simulink model "MPPT_PO1"  (R2024b)
settings: Solver=ode45  StartTime=0.0  StopTime=10.0  MaxStep=1e-4  RelTol=1e-3
libraries: powerlib_extras x2, simulink x1, spspowerguiLib x1
settings Model: Creator=Abdo  LastModifiedBy=Eng.Abd-Elrhman Saad
settings SolverCC: ZeroCrossAlgorithm=Adaptive  AlgebraicLoopSolver=TrustRegion
settings DataIOCC: SaveFormat=StructureWithTime  ReturnWorkspaceOutputs=off
settings OptimizationCC: LifeSpan=inf
settings DebuggingCC: MaxConsecutiveZCsMsg=none  UnconnectedInputMsg=warning  UnconnectedOutputMsg=warning  UnconnectedLineMsg=warning  SFExecutionAtInitializationDiag=none  ArithmeticOperatorsInVariantConditions=warning
settings HardwareCC: ProdBitPerSizeT=32  ProdBitPerPtrDiffT=32  ProdWordSize=32  ProdHWDeviceType=Specified
settings SFSimCC: SimUseLocalCustomCode=off  CustomCodeUndefinedFunction=UseInterfaceOnly
settings RTWCC: RTWUseLocalCustomCode=off  GPUComputeCapability=3.5
settings CodeAppCC: StateflowObjectComments=on

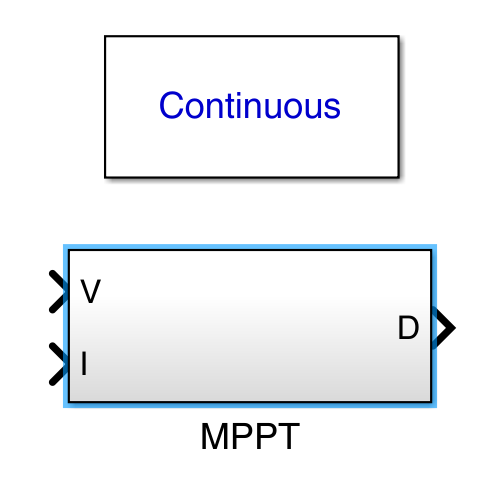
[thumbnail: Simulink's stored preview of the top-level diagram]
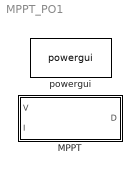
== system MPPT_PO1 ==
  MPPT : Subsystem
  powergui : spspowerguiLib/powergui  Priority=1  SimulationMode=Continuous  SampleTime=50e-6  frequency=60  Iterations=50  frequencyindice=0  Pbase=100e6  ErrMax=1e-4  UnitsV=kV  UnitsW=MW  buscounter=0  FunctionMessages=off  echomessages=off  EnableUseOfTLC=off  CurrentSourceSwitches=off  DisableSnubberDevices=off  DisableRonSwitches=off  DisableVfSwitches=off  DisplayEquations=off  AutomaticDiscreteSolvers=off  SolverType=Tustin/Backward Euler (TBE)  Interpol=off  ExternalGateDelay=off  methode=off  Ts=100  x0status=blocks  SPID=on  SwTol=0  HookPort=off  NonlinearTolerance=1e-4  nMaxIteration=100  ContinueOnMaxIteration=off  RestoreLinks=warning  ResistiveCurrentMeasurement=off  Frange=[0:2:500]  Ylog=off  Xlog=on  ShowGrid=off  save=off  variable=ZData  structure=0  ZoomFFT=off  StartTime=0.0  cycles=1  DisplayStyle=1  fundamental=60  FreqAxis=off  MaxFrequency=1000  frequencyindicesteady=1  RmsSteady=1  display=off

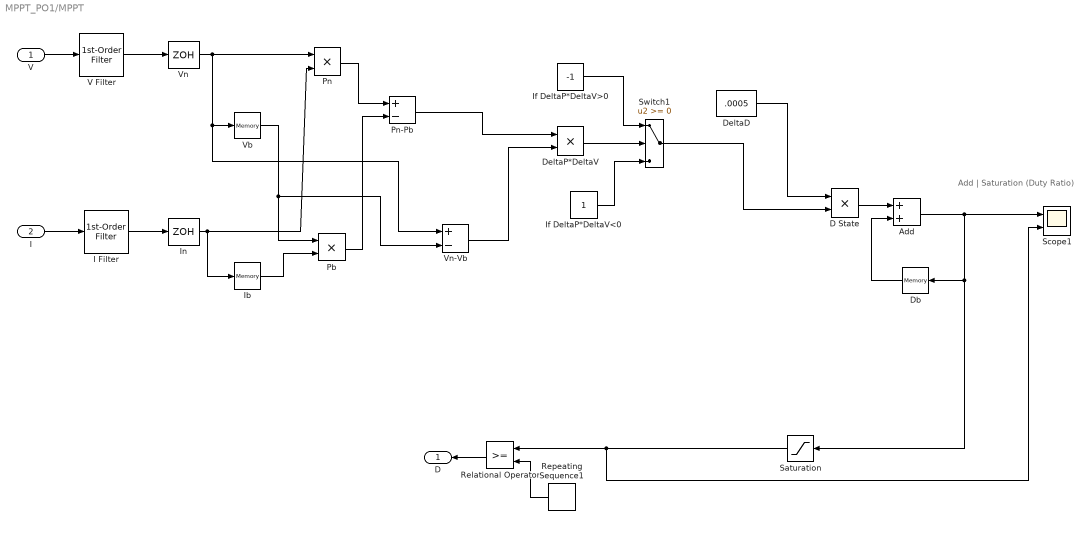
== system MPPT_PO1/MPPT ==
  note: Add | Saturation (Duty Ratio)
  V : Inport
  I : Inport  Port=2
  Add : Sum
  D State : Product  RndMeth=Zero
  Db : Memory  InheritSampleTime=on  LinearizeAsDelay=on
  DeltaD : Constant  Value=.0005
  DeltaP*DeltaV : Product  RndMeth=Zero
  I Filter : powerlib_extras/Control  Blocks/1st-Order  Filter  FilterType=Lowpass  Tc=1e-3  Initialize=off  Vac_Init=[0.8 -25 60]  Vdc_Init=-0.4  PlotResponse=off  param1=[1 500 1]
  Ib : Memory  InheritSampleTime=on  LinearizeAsDelay=on
  If DeltaP*DeltaV<0 : Constant
  If DeltaP*DeltaV>0 : Constant  Value=-1
  In : ZeroOrderHold  SampleTime=1e-4
  Pb : Product  RndMeth=Zero
  Pn : Product  RndMeth=Zero
  Pn-Pb : Sum  Inputs=+-
  Relational Operator : RelationalOperator  OutDataTypeStr=boolean  InputSameDT=off
  Repeating Sequence1 : simulink/Sources/Repeating Sequence  rep_seq_t=[0 1e-3]  rep_seq_y=[0 1]
  Saturation : Saturate  UpperLimit=0.9  LowerLimit=0
  Scope1 : Scope  NumInputPorts=2
  Switch1 : Switch  SaturateOnIntegerOverflow=off  InputSameDT=off
  V Filter : powerlib_extras/Control  Blocks/1st-Order  Filter  FilterType=Lowpass  Tc=1e-3  Initialize=off  Vac_Init=[0.8 -25 60]  Vdc_Init=-0.4  PlotResponse=off  param1=[1 500 1]
  Vb : Memory  InheritSampleTime=on  LinearizeAsDelay=on
  Vn : ZeroOrderHold  SampleTime=1e-4
  Vn-Vb : Sum  Inputs=+-
  D : Outport
  wires:
  V/1 -> V Filter/1
  I/1 -> I Filter/1
  V Filter/1 -> Vn/1
  I Filter/1 -> In/1
  In/1 -> Ib/1, Pn/2
  Vn/1 -> Pn/1, Vb/1, Vn-Vb/1
  Ib/1 -> Pb/2
  Vb/1 -> Pb/1, Vn-Vb/2
  Pn/1 -> Pn-Pb/1
  Pb/1 -> Pn-Pb/2
  D State/1 -> Add/1
  Repeating Sequence1/1 -> Relational Operator/2
  Relational Operator/1 -> D/1
  Db/1 -> Add/2
  Add/1 -> Saturation/1, Db/1, Scope1/1
  Pn-Pb/1 -> DeltaP*DeltaV/1
  Vn-Vb/1 -> DeltaP*DeltaV/2
  DeltaP*DeltaV/1 -> Switch1/2
  If DeltaP*DeltaV>0/1 -> Switch1/1
  If DeltaP*DeltaV<0/1 -> Switch1/3
  Switch1/1 -> D State/2
  DeltaD/1 -> D State/1
  Saturation/1 -> Relational Operator/1, Scope1/2
